simulink model "modele_qpsk_filtre"  (R2024b)
settings: Solver=FixedStepDiscrete  StartTime=0.0  StopTime=(Nsim-1)*Tb  FixedStep=Te  RelTol=1e-3
values from neighbouring files (symbols this model uses):
  L = @(a, b) add_line(blk, a, b, 'autorouting', 'on')    [ajouter_codeur_registre.m]    (also in ajouter_decodeur_hamming.m; ajouter_modem_qpsk.m; ajouter_modem_qpsk_filtre.m; construire_modele_codeur_registre.m = @(a, b) add_line(mdl, a, b, 'autorouting', 'on'))
undefined symbols (not defined in the file or in its folder): dPhase, graine, hE, N0, Tb, Te
settings Model: Creator=youka  LastModifiedBy=youka

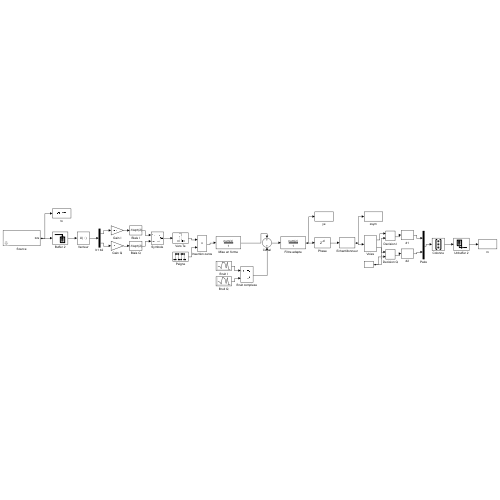
[thumbnail: Simulink's stored preview of the top-level diagram]
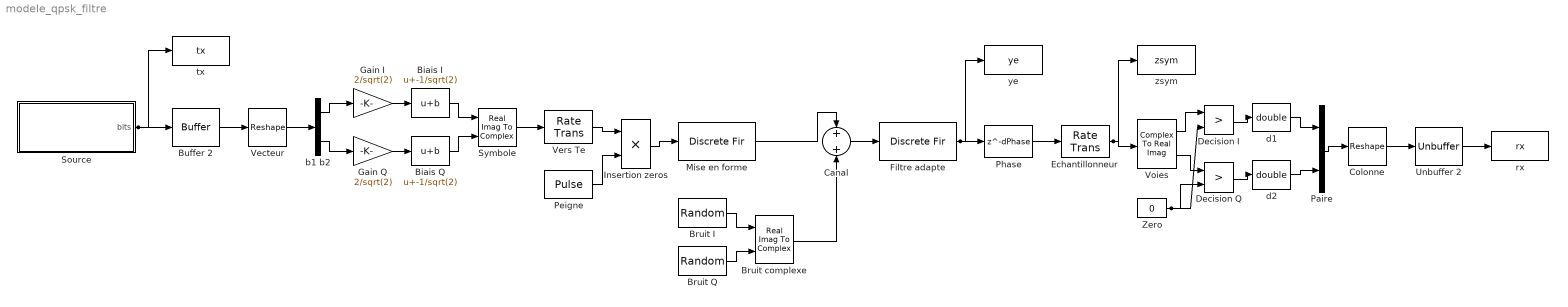
== system modele_qpsk_filtre ==
  Biais I : Bias  Bias=-1/sqrt(2)  SaturateOnIntegerOverflow=off
  Biais Q : Bias  Bias=-1/sqrt(2)  SaturateOnIntegerOverflow=off
  Bruit I : RandomNumber  Variance=N0/2  Seed=graine+1  SampleTime=Te
  Bruit Q : RandomNumber  Variance=N0/2  Seed=graine+2  SampleTime=Te
  Bruit complexe : RealImagToComplex
  Buffer 2 : Buffer  N=2
  Canal : Sum
  Colonne : Reshape  OutputDimensionality=Column vector (2-D)
  Decision I : RelationalOperator  Operator=>  OutDataTypeStr=boolean  RndMeth=Simplest  InputSameDT=off
  Decision Q : RelationalOperator  Operator=>  OutDataTypeStr=boolean  RndMeth=Simplest  InputSameDT=off
  Echantillonneur : RateTransition  OutPortSampleTime=Ts
  Filtre adapte : DiscreteFir  Coefficients=fliplr(hE)
  Gain I : Gain  Gain=2/sqrt(2)
  Gain Q : Gain  Gain=2/sqrt(2)
  Insertion zeros : Product  Inputs=**
  Mise en forme : DiscreteFir  Coefficients=hE
  Paire : Mux  Inputs=2
  Peigne : DiscretePulseGenerator  Period=L  SampleTime=Te
  Phase : Delay  DelayLength=dPhase
  Source : Subsystem  mask(Source binaire){p_m=0.5, Tb_m=Tb, graine_m=graine}
      mask prompts: p_m "Probabilité d'émettre un 1"; Tb_m "Durée d'un bit Tb (s)"; graine_m "Graine (Seed)"
      mask help: Source binaire sans mémoire : P(1) = p, un bit toutes les Tb secondes.
  Symbole : RealImagToComplex
  Unbuffer 2 : Unbuffer
  Vecteur : Reshape
  Vers Te : RateTransition  OutPortSampleTime=Te
  Voies : ComplexToRealImag
  Zero : Constant  Value=0
  b1 b2 : Demux  Outputs=2
  d1 : DataTypeConversion  OutDataTypeStr=double  SaturateOnIntegerOverflow=off  RndMeth=Floor
  d2 : DataTypeConversion  OutDataTypeStr=double  SaturateOnIntegerOverflow=off  RndMeth=Floor
  rx : ToWorkspace  VariableName=rx  SampleTime=-1
  tx : ToWorkspace  VariableName=tx  SampleTime=-1
  ye : ToWorkspace  VariableName=ye  SampleTime=-1
      settings: MaxDataPoints=Nlog
  zsym : ToWorkspace  VariableName=zsym  SampleTime=-1
  wires:
  Source/1(bits) -> tx/1, Buffer 2/1
  Buffer 2/1 -> Vecteur/1
  Vecteur/1 -> b1 b2/1
  b1 b2/1 -> Gain I/1
  Gain I/1 -> Biais I/1
  Biais I/1 -> Symbole/1
  b1 b2/2 -> Gain Q/1
  Gain Q/1 -> Biais Q/1
  Biais Q/1 -> Symbole/2
  Symbole/1 -> Vers Te/1
  Vers Te/1 -> Insertion zeros/1
  Peigne/1 -> Insertion zeros/2
  Insertion zeros/1 -> Mise en forme/1
  Bruit I/1 -> Bruit complexe/1
  Bruit Q/1 -> Bruit complexe/2
  Mise en forme/1 -> Canal/1
  Bruit complexe/1 -> Canal/2
  Canal/1 -> Filtre adapte/1
  Filtre adapte/1 -> ye/1, Phase/1
  Phase/1 -> Echantillonneur/1
  Echantillonneur/1 -> zsym/1, Voies/1
  Voies/1 -> Decision I/1
  Zero/1 -> Decision I/2, Decision Q/2
  Voies/2 -> Decision Q/1
  Decision I/1 -> d1/1
  Decision Q/1 -> d2/1
  d1/1 -> Paire/1
  d2/1 -> Paire/2
  Paire/1 -> Colonne/1
  Colonne/1 -> Unbuffer 2/1
  Unbuffer 2/1 -> rx/1

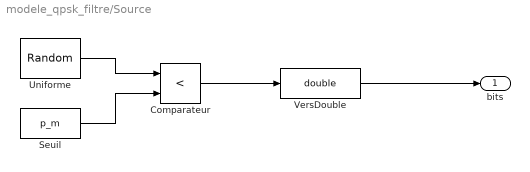
== system modele_qpsk_filtre/Source ==
  Comparateur : RelationalOperator  Operator=<  OutDataTypeStr=boolean  RndMeth=Simplest  InputSameDT=off
  Seuil : Constant  Value=p_m  SampleTime=Tb_m
  Uniforme : UniformRandomNumber  Minimum=0  Seed=graine_m  SampleTime=Tb_m
  VersDouble : DataTypeConversion  OutDataTypeStr=double  SaturateOnIntegerOverflow=off  RndMeth=Floor
  bits : Outport
  wires:
  Uniforme/1 -> Comparateur/1
  Seuil/1 -> Comparateur/2
  Comparateur/1 -> VersDouble/1
  VersDouble/1 -> bits/1
